simulink model "arducopter"  (R2024b)
settings: Solver=FixedStepAuto  StartTime=0.0  StopTime=simIn.param.timeEnd  FixedStep=simIn.param.dt  RelTol=1e-3
undefined symbols (not defined in the file or in its folder): DiscIntNeverNeededParam, sim, simIn
libraries: simulink x60, slident x4, vrlib x1
(part 8 of 9)

== matlab function arducopter/Rate Controller/PID Yaw Rate/Slew Limiter/Calculate Dmod ==
  data: slew_rate input; Dmod output single; sr_max input; sr_tau input; dt input; time input; pos_event_idx data_store_memory; pos_event_stored data_store_memory; pos_event_ms data_store_memory; neg_event_idx data_store_memory; neg_event_stored data_store_memory; neg_event_ms data_store_memory; modifier_slew_rate data_store_memory; output_slew_rate data_store_memory; max_neg_slew_event_ms data_store_memory; max_pos_slew_event_ms data_store_memory; max_neg_slew_rate data_store_memory; max_pos_slew_rate data_store_memory
function Dmod   = fcn(slew_rate, sr_max, sr_tau, dt, time)
% Code is based on SlewLimiter::modifier() in SlewLimiter.cpp. 

% Define global variables, so that quanitities do not have to be fed back
% to the function
global pos_event_stored;
global pos_event_idx;
global pos_event_ms;
global max_pos_slew_rate;
global max_pos_slew_event_ms;
global neg_event_stored;
global neg_event_idx;
global neg_event_ms;
global max_neg_slew_rate;
global max_neg_slew_event_ms;
global modifier_slew_rate;
global output_slew_rate;

% Definition of constants as done in SlewLimiter.h
SLEWLIMITER_N_EVENTS = uint32(3); % Number of positive and negative consecutive slew rate exceedance events recorded. Set to 3 because of 1-based indexing.
WINDOW_MS = uint32(300); % Time in ms required for half a cycle of the slowest oscillation frequency expected
MODIFIER_GAIN = 1.5; % Ratio of modifier reduction to slew rate exceedance

if (dt < 0)
    Dmod = single(1.0);
    return;
end

now_ms = uint32(time);
decay_alpha = min(dt, sr_tau) / sr_tau;

% Apply a filter to decay maximum seen slew rate once the value had left the window period
attack_alpha = min(2.0 * decay_alpha, 1.0);

%% Calculate maximum slew rate
% Save new maximum slew rates, if oldest maximum is exceeded
% OR decay the peak slew rates (pos. and neg.) if they are outside the
% observed time window
% Never drop PID gains below 10% of configured value
if (slew_rate > max_pos_slew_rate)
    max_pos_slew_rate(:) = slew_rate;
    max_pos_slew_event_ms = now_ms;
elseif (now_ms - max_pos_slew_event_ms > WINDOW_MS)
    max_pos_slew_rate = max_pos_slew_rate * (1.0 - decay_alpha);
end

if (-slew_rate > max_neg_slew_rate)
    max_neg_slew_rate(:) = -slew_rate;
    max_neg_slew_event_ms = now_ms;
elseif (now_ms - max_neg_slew_event_ms > WINDOW_MS)
    max_neg_slew_rate = max_neg_slew_rate * (1.0 - decay_alpha);
end

% Calculate the averaged maximum slew rate
raw_slew_rate = 0.5 * (max_pos_slew_rate + max_neg_slew_rate);
% Calculation of output slew rate
output_slew_rate = output_slew_rate + (raw_slew_rate - output_slew_rate) * attack_alpha;
output_slew_rate = min(raw_slew_rate, output_slew_rate);

% Check if slew limiter is activated
if(sr_max <= 0)
   Dmod = single(1.0);
   return;
end

% Constrain slew rate used for calculation
limited_raw_slew_rate = 0.5 * (min(max_pos_slew_rate, 10 * sr_max) + min(max_neg_slew_rate, 10 * sr_max));


%% Save exceedance events in event time vector
% Store a series of positive slew rate exceedance events
if (~pos_event_stored && slew_rate > sr_max)
    if (pos_event_idx >= SLEWLIMITER_N_EVENTS)
        pos_event_idx(:) = 1;
    end
    pos_event_ms(pos_event_idx) = now_ms;
    pos_event_idx(:) = pos_event_idx + 1;
    pos_event_stored = true;
    neg_event_stored = false;
end

% Store a series of negative slew rate exceedance events
if (~neg_event_stored && -slew_rate > sr_max)
    if (neg_event_idx >= SLEWLIMITER_N_EVENTS)
        neg_event_idx(:) = 1;
    end
    neg_event_ms(neg_event_idx) = now_ms;
    neg_event_idx(:) = neg_event_idx + 1;
    pos_event_stored = false;
    neg_event_stored = true;
end

% Find oldest event time
oldest_ms = now_ms;
for i=1:SLEWLIMITER_N_EVENTS-1
   oldest_ms = min(oldest_ms, pos_event_ms(i));
   oldest_ms = min(oldest_ms, neg_event_ms(i));
end

% When the oldest exceedance event falls outside of the window required for
% the number of exceedance events, apply a further reduction to the maximum
% slew rate. This prevents unwanted gain reductions caused by spikes in the
% demanded angular rates due to changed control modes or similar causes.
modifier_input = limited_raw_slew_rate;
if(now_ms - oldest_ms > SLEWLIMITER_N_EVENTS * WINDOW_MS) % no incrementation of SLEWLIMITER_N_EVENTS because of 1 based indexing
   oldest_time_from_window = single(0.001) * single(now_ms - oldest_ms - SLEWLIMITER_N_EVENTS * WINDOW_MS); 
   modifier_input = modifier_input * single(exp(-oldest_time_from_window / sr_tau));
end

%% Calculation of modifier slew rate

modifier_slew_rate = modifier_slew_rate + (modifier_input - modifier_slew_rate) * attack_alpha;
modifier_slew_rate = min(modifier_slew_rate, modifier_input);

% Calculate modifier. Only has an impact if sr_max is exceeded by averaged
% slew rate.
if(modifier_slew_rate > sr_max)
    Dmod(:) = sr_max / (sr_max + MODIFIER_GAIN * (modifier_slew_rate - sr_max));
else
    Dmod(:) = 1.0;
end

== matlab function arducopter/Position Controller/PID Velocity z/I/Integrator ==
  data: error input; integrator_out output; integrator input single; limitNeg input; limitPos input; ki input; i_max input; dt input
function integrator_out = fcn(error, integrator, limitNeg, limitPos, ki, i_max, dt)
% Code is based on AC_PID_Basic::update_i() in AC_PID_Basic.

% Check plausibility of input parameters
if (ki ~= 0)
    % Integration can only be executed if limits are not exceeded or if
    % limits are exceeded but the current error would reduce output
    if (~((limitNeg && error < 0) || (limitPos && error > 0)))
        integrator_out = integrator + error * ki * dt;
        integrator_out = max( min(integrator_out, i_max), -i_max);
    else % Otherwise, keep old integrator value
        integrator_out = integrator;
    end
else % Reset integrator if input parameters are not plausible
    integrator_out = single(0.0);
end

== matlab function arducopter/Position Controller/PID Acceleration z/I/Integrator ==
  data: error input; integrator_out output; integrator input single; limit_flg input; ki input; i_max input; dt input
function integrator_out = fcn(error, integrator, limit_flg, ki, i_max, dt)
% Code is based on AC_PID::update_i() in AC_PID, line 230.

% Check plausibility of input parameters
if (ki ~= 0 && dt > 0)
    % Only allow integration if limit is not set or the absolute sum of the
    % integrator would be reduced.
    if (~limit_flg || (integrator > 0 && error < 0) || (integrator < 0 && error > 0))
        integrator_out = integrator + error * ki * dt;
        integrator_out = min( max(integrator_out, -i_max), i_max);
    else % Otherwise, keep old integrator value
        integrator_out = integrator;
    end
else % Reset integrator if input parameters are not plausible
    integrator_out = single(0.0);
end

== matlab function arducopter/Position Controller/PID Acceleration z/Slew Limiter/Calculate Dmod ==
  data: slew_rate input; Dmod output single; sr_max input; sr_tau input; dt input; time input; pos_event_idx data_store_memory; pos_event_stored data_store_memory; pos_event_ms data_store_memory; neg_event_idx data_store_memory; neg_event_stored data_store_memory; neg_event_ms data_store_memory; modifier_slew_rate data_store_memory; output_slew_rate data_store_memory; max_neg_slew_event_ms data_store_memory; max_pos_slew_event_ms data_store_memory; max_neg_slew_rate data_store_memory; max_pos_slew_rate data_store_memory
function Dmod   = fcn(slew_rate, sr_max, sr_tau, dt, time)
% Code is based on SlewLimiter::modifier() in SlewLimiter.cpp. 

% Define global variables, so that quanitities do not have to be fed back
% to the function
global pos_event_stored;
global pos_event_idx;
global pos_event_ms;
global max_pos_slew_rate;
global max_pos_slew_event_ms;
global neg_event_stored;
global neg_event_idx;
global neg_event_ms;
global max_neg_slew_rate;
global max_neg_slew_event_ms;
global modifier_slew_rate;
global output_slew_rate;

% Definition of constants as done in SlewLimiter.h
SLEWLIMITER_N_EVENTS = uint32(3); % Number of positive and negative consecutive slew rate exceedance events recorded. Set to 3 because of 1-based indexing.
WINDOW_MS = uint32(300); % Time in ms required for half a cycle of the slowest oscillation frequency expected
MODIFIER_GAIN = 1.5; % Ratio of modifier reduction to slew rate exceedance

if (dt < 0)
    Dmod = single(1.0);
    return;
end

now_ms = uint32(time);
decay_alpha = min(dt, sr_tau) / sr_tau;

% Apply a filter to decay maximum seen slew rate once the value had left the window period
attack_alpha = min(2.0 * decay_alpha, 1.0);

%% Calculate maximum slew rate
% Save new maximum slew rates, if oldest maximum is exceeded
% OR decay the peak slew rates (pos. and neg.) if they are outside the
% observed time window
% Never drop PID gains below 10% of configured value
if (slew_rate > max_pos_slew_rate)
    max_pos_slew_rate(:) = slew_rate;
    max_pos_slew_event_ms = now_ms;
elseif (now_ms - max_pos_slew_event_ms > WINDOW_MS)
    max_pos_slew_rate = max_pos_slew_rate * (1.0 - decay_alpha);
end

if (-slew_rate > max_neg_slew_rate)
    max_neg_slew_rate(:) = -slew_rate;
    max_neg_slew_event_ms = now_ms;
elseif (now_ms - max_neg_slew_event_ms > WINDOW_MS)
    max_neg_slew_rate = max_neg_slew_rate * (1.0 - decay_alpha);
end

% Calculate the averaged maximum slew rate
raw_slew_rate = 0.5 * (max_pos_slew_rate + max_neg_slew_rate);
% Calculation of output slew rate
output_slew_rate = output_slew_rate + (raw_slew_rate - output_slew_rate) * attack_alpha;
output_slew_rate = min(raw_slew_rate, output_slew_rate);

% Check if slew limiter is activated
if(sr_max <= 0)
   Dmod = single(1.0);
   return;
end

% Constrain slew rate used for calculation
limited_raw_slew_rate = 0.5 * (min(max_pos_slew_rate, 10 * sr_max) + min(max_neg_slew_rate, 10 * sr_max));


%% Save exceedance events in event time vector
% Store a series of positive slew rate exceedance events
if (~pos_event_stored && slew_rate > sr_max)
    if (pos_event_idx >= SLEWLIMITER_N_EVENTS)
        pos_event_idx(:) = 1;
    end
    pos_event_ms(pos_event_idx) = now_ms;
    pos_event_idx(:) = pos_event_idx + 1;
    pos_event_stored = true;
    neg_event_stored = false;
end

% Store a series of negative slew rate exceedance events
if (~neg_event_stored && -slew_rate > sr_max)
    if (neg_event_idx >= SLEWLIMITER_N_EVENTS)
        neg_event_idx(:) = 1;
    end
    neg_event_ms(neg_event_idx) = now_ms;
    neg_event_idx(:) = neg_event_idx + 1;
    pos_event_stored = false;
    neg_event_stored = true;
end

% Find oldest event time
oldest_ms = now_ms;
for i=1:SLEWLIMITER_N_EVENTS-1
   oldest_ms = min(oldest_ms, pos_event_ms(i));
   oldest_ms = min(oldest_ms, neg_event_ms(i));
end

% When the oldest exceedance event falls outside of the window required for
% the number of exceedance events, apply a further reduction to the maximum
% slew rate. This prevents unwanted gain reductions caused by spikes in the
% demanded angular rates due to changed control modes or similar causes.
modifier_input = limited_raw_slew_rate;
if(now_ms - oldest_ms > SLEWLIMITER_N_EVENTS * WINDOW_MS) % no incrementation of SLEWLIMITER_N_EVENTS because of 1 based indexing
   oldest_time_from_window = single(0.001) * single(now_ms - oldest_ms - SLEWLIMITER_N_EVENTS * WINDOW_MS); 
   modifier_input = modifier_input * single(exp(-oldest_time_from_window / sr_tau));
end

%% Calculation of modifier slew rate

modifier_slew_rate = modifier_slew_rate + (modifier_input - modifier_slew_rate) * attack_alpha;
modifier_slew_rate = min(modifier_slew_rate, modifier_input);

% Calculate modifier. Only has an impact if sr_max is exceeded by averaged
% slew rate.
if(modifier_slew_rate > sr_max)
    Dmod(:) = sr_max / (sr_max + MODIFIER_GAIN * (modifier_slew_rate - sr_max));
else
    Dmod(:) = 1.0;
end

== matlab function arducopter/Motor Mixer/Calculate motor thrust ==
  data: roll input; limitRoll output; limitPitch output; pitch input; yaw input; thrIn input; thrAvgMax input; thrThstMaxIn input; compGain input; yawHeadroom input; numMotors input; facMotors input; limitYaw output; limitThrLower output; limitThrUpper output; thrOut output; thstOut output; thst_rpyt data_store_memory
function [limitRoll, limitPitch, limitYaw, limitThrLower, limitThrUpper, thrOut, thstOut] = outputArmedStabilizing(roll, pitch, yaw, thrIn, thrAvgMax, thrThstMaxIn, compGain, yawHeadroom, numMotors, facMotors)
% The calculation is taken from output_armed_stabilizing() in
% AP_MotorsMatrix.cpp.
% Contrary to the original code, lost motors are not considered

global thst_rpyt;

%% Preperations
% Definitions
roll_factor = facMotors(1,:);              % Factors of motors for thrust on differen axis - needs to moved to Init-file, together with calculation
pitch_factor = facMotors(2,:);
yaw_factor = facMotors(3,:);
throttle_factor = facMotors(4,:);
limitRoll = false;                             % Initialize limit flags to prevent missing assignment error of Simulink
limitPitch = false;
limitYaw = false;
limitThrLower = false;
limitThrUpper = false;
yaw_allowed = single(1.0);                          % Amount of yaw that can be realized
rpy_scale = single(1.0);                            % Scale factor to fit roll, pitch and yaw within motor limits
throttle_thrust_best_rpy = single(0.0);             % Amount of throttle that provides maximum roll, pitch and yaw without climbing                      
thrust_boost_ratio = single(0.0);                   % Ratio for thrust boosting in case of a motor failure. Set to 0 for normal operation!     

% TODO: Voltage and air pressure compensation
roll_thrust = roll * compGain;
pitch_thrust = pitch * compGain;
yaw_thrust = yaw * compGain;
throttle_thrust = thrIn * compGain;             % Pilot's desired throttle
thrAvgMax = thrAvgMax * compGain;

% Calculate maximum throttle thrust input value
throttle_thrust_max = thrust_boost_ratio + (1.0 - thrust_boost_ratio) * thrThstMaxIn;

% Sanity check: Throttle above zero and below current limnited throttle.
% Limit Throttle otherwise
if (throttle_thrust <= 0)
    throttle_thrust = single(0.0);
    limitThrLower = true;
end
if (throttle_thrust >= throttle_thrust_max)
    throttle_thrust = throttle_thrust_max;
    limitThrUpper = true;
end
% Limit throttle average max
thrAvgMax = max( min( thrAvgMax, throttle_thrust_max), throttle_thrust);
% Calculate highest allowed average throttle that will provide maximum
% control range of roll, pitch and yaw without climbing
throttle_thrust_best_rpy = min(single(0.5), thrAvgMax);

%% Calculation of the throttle that gives most room for yaw
% This corresponds to the lower of
%   1. 0.5 - (rpy_low + rpy_high) / 2.0) --> This gives the maximum
%   possible margin above the highest motor and below the lowest
%   2. The higher of
%       a) Pilots throttle input
%       b) The point throttle_rpy_mix between pilot's input throttle and
%       hover throttle

% First: Calculate amount of yaw that fits into throttle range
% amount of yaw we can fit in
yaw_allowed = single(1.0);
for i=1:numMotors
    % Combined thrust output of roll and pitch
    thst_rpyt(i) = roll_thrust * roll_factor(i) + pitch_thrust * pitch_factor(i); 
    
    % % Record lowest thrust command
    % if (thst_rpyt(i) < rp_low)
    %     rp_low = thst_rpyt(i);
    % end
    % % Record highest thrust command
    % if (thst_rpyt(i) > rp_high)
    %     rp_high = thst_rpyt(i);
    % end
    
    % Check maximum yaw control that can be used
    if(yaw_factor(i)~=0)
        thrust_rp_best_throttle = throttle_thrust_best_rpy + thst_rpyt(i);
        if ((yaw_thrust * yaw_factor(i)) > 0)
           motor_room = 1 - thrust_rp_best_throttle;
        else
           motor_room = thrust_rp_best_throttle;
        end
        motor_yaw_allowed = max(motor_room, 0) / abs(yaw_factor(i));
        yaw_allowed = min(yaw_allowed, motor_yaw_allowed);
    end    
end

% Calculate the maximum yaw control that can be used
yaw_allowed_min = yawHeadroom / 1000.0;
% If thrust boost is enabled, increase headroom to 50%
yaw_allowed_min = thrust_boost_ratio * 0.5 + (1.0 - thrust_boost_ratio) * yaw_allowed_min;

yaw_allowed = max(yaw_allowed, yaw_allowed_min);

%% Add yaw control to thrust outputs
% Limit yaw thrust to allowed range
if (abs(yaw_thrust) > yaw_allowed)
    yaw_thrust = min( max(-yaw_allowed, yaw_thrust), yaw_allowed);
    limitYaw = true;
end

rpy_low = single(1.0);
rpy_high = single(-1.0);
for i=1:numMotors
    % Combined thrust command for roll, pitch and yaw
   thst_rpyt(i) = thst_rpyt(i) + yaw_thrust * yaw_factor(i);
   
   % Record lowest thrust command
    if (thst_rpyt(i) < rpy_low)
        rpy_low = thst_rpyt(i);
    end
    % Record highest thrust command
    if (thst_rpyt(i) > rpy_high)
        rpy_high = thst_rpyt(i);
    end
end

%% Scale outputs
% Calculate any sclaing that is needed to fit combined thrust outputs
% within the output range
if (rpy_high - rpy_low > 1.0)
    rpy_scale(:) = 1.0 / (rpy_high-rpy_low);
end
if (thrAvgMax + rpy_low < 0)
    rpy_scale(:) = min(rpy_scale, -thrAvgMax / rpy_low);
end

% Calculate how close the motors can come to the desired throttle
rpy_high = rpy_high * rpy_scale;
rpy_low = rpy_low * rpy_scale;
throttle_thrust_best_rpy = -rpy_low;
% Calculate the difference between pilot's desired throttle and
% throttle_thrust_best_rpy
thr_adj = single(throttle_thrust - throttle_thrust_best_rpy);
if (rpy_scale < 1.0) % Full range of throttle is already being used
    limitRoll(:) = true;
    limitPitch(:) = true;
    limitYaw(:) = true;
    if (thr_adj > 0.0)
       limitThrUpper = true; 
    end
    thr_adj(:) = 0.0;
else
    if (thr_adj < 0.0) % Throttle can't be reduced to reach desired value
        thr_adj(:) = 0.0;
    elseif (thr_adj > 1.0 - (throttle_thrust_best_rpy + rpy_high))
       % Throttle can't be increased to desired value
       thr_adj(:) = 1.0 - (throttle_thrust_best_rpy + rpy_high);
       limitThrUpper = true;
    end
end

%% Calculate resulting thrust outputs
% Calculate adjusted throttle value
throttle_thrust_best_plus_adj = throttle_thrust_best_rpy + thr_adj;
% Add scaled roll, pitch, constrained yaw and throttle for each motor
for i=1:numMotors
    % Combined thrust is the sum of the maximum possible desired throttle
    % "throttle_thrust_best_plus_adj" and the needed thrust to realize the
    % desired angular motion "thrust_rpyt_out(i)"
    thst_rpyt(i) = (throttle_thrust_best_plus_adj * throttle_factor(i)) + (rpy_scale * thst_rpyt(i)); 
end

% Calculate throttle thrust after mixing for harmonic notch
thrOut = throttle_thrust_best_plus_adj / compGain;

% Assign thrust output
thstOut = thst_rpyt;

== matlab function arducopter/Position Controller/P Position z/Calculate error ==
  settings: updateMethod=DISCRETE
  data: tar input; tar_new output; err output; act input; err_min input; err_max input
function [tar_new, err] = calc_err(tar, act, err_min, err_max)
% Code based on AC_P_1D::update_all() in AC_P_1D.cpp.
tar_new = tar; % added line to prevent Simulink error for unassigned tar_new
err = tar - act;

% Limit error and recalculate target
if ((err_min < 0) && (err < err_min))
    err = err_min;
    tar_new = act + err;
elseif ((err_max > 0) && (err > err_max))
    err = err_max;
    tar_new = act + err;
end

== matlab function arducopter/Position Controller/P Position z/Set vertical speed & acceleration limit/Set error limits ==
  data: outMin input; errMin output; outMax input; DoutMax input; errMax output; D1max output; D2OutMax input; kp input
function [errMin, errMax, D1max] = setLimits(outMin, outMax, DoutMax, D2OutMax, kp)
% Code taken from AC_P_1D::set_limits() in AC_P_1D.cpp.
% Input parameter D2_out_max is neglected since it is set to zero in
% AC_PosControl::set_correction_speed_accel_z()

errMin = single(0.0);
errMax = single(0.0);
D1max = single(0.0);

if (DoutMax > 0)
   D1max = DoutMax; 
end

% Missing line left out because of parameter D2_out_max being set to 0

% Call the simulink function inv_sqrt_controller(...) from control.cpp,
% line 343 if the conditions apply
if (outMin < 0 && kp > 0)
    errMin = inv_sqrt_controller(outMin, kp, DoutMax);
end

if (outMax > 0 && kp > 0)
    errMax = inv_sqrt_controller(outMax, kp, DoutMax);
end

== matlab function arducopter/Position Controller/P Position z/Set vertical speed & acceleration limit/Inverse Square Root Controller/Inverse Sqrt Controller ==
  data: output input; errLim output; p input; Dmax input
function errLim = inv_sqrt_controller(output, p, Dmax)
% Code taken from inv_sqrt_controller(...) in control.cpp.
% Function calculates the input (error) to the sqrt_controller required to
% achieve a given output

if (Dmax > 0 && p == 0)
    errLim = output * output / (single(2.0) * Dmax);
    return;
end
if ((Dmax < 0 || Dmax == 0) && p ~= 0)
    errLim = output / p;
    return;
end
if ((Dmax < 0 || Dmax == 0) && p == 0)
   errLim = single(0.0);
   return
end

% Calculate the cross-point velocity, at which we switch from calculating the
% controller output using a linear function to a sqrt function
linear_velocity = Dmax / p;
% Use linear function to calculate limit if current velocity is below
% cross-point velocity
if (abs(output) < linear_velocity)
   errLim = output / p;
   return;
end

% Calculate the cross-point distance at which we switch to sqrt function
linear_dist = Dmax / (p*p);
% Calculate the maximum distance error resulting from the velocity and
% acceleration limit
stopping_dist = (linear_dist * single(0.5)) + (output*output) / (single(2.0) * Dmax);
% If output parameter is negative or zero, return negative maximum distance
% error
if (output > 0)
    errLim = stopping_dist;
else
    errLim = -stopping_dist;
end

== matlab function arducopter/Position Controller/P Position z/Square Root Controller ==
  data: err input; correction_rate output; p input; second_ord_lim input; dt input
function correction_rate = sqrt_controller(err, p, second_ord_lim, dt)
% The square root controller
% Code is taken from sqrt_controller(...) in AC_PosControl.cpp.

if (second_ord_lim < 0 || second_ord_lim == 0)
   correction_rate = err * p;
elseif (p == 0)
    % P term is zero, but second order limit is positive
    if (err > 0)
        correction_rate = sqrt(single(2.0) * second_ord_lim * err);
    elseif (err < 0)
        correction_rate = sqrt(single(2.0) * second_ord_lim * -err);
    else
        correction_rate = single(0.0);
    end
else
    % P term and second order limit are positive, hence have been defined
    linear_dist = second_ord_lim / (p * p);
    % Check if error exceeds linear range of controller gain
    if (err > linear_dist)
        correction_rate = sqrt(single(2.0) * second_ord_lim * ( err - (linear_dist / single(2.0)) ));
    elseif (err < -linear_dist)
        correction_rate = -sqrt(single(2.0) * second_ord_lim * ( -err - (linear_dist / single(2.0)) ));
    else
        % Return linearly amplified correction if error is in linear range
        correction_rate = err * p;
    end
end

% Prevent oscillations by over-shooting the error correction in the last
% time step
if (dt > 0)
    correction_rate = min( max(correction_rate, -abs(err) / dt), abs(err) / dt);
end

== matlab function arducopter/Position Controller/PID Acceleration z/Slew Limiter/Lowpass Filter ==
  data: in input; out output single; alpha input; out_last input
function out  = apply(in, alpha, out_last)
% The code is based on the apply(sample, cutoff_freq, dt) function in
% LowPassFilter.cpp

% Output calculation
out = out_last + (in - out_last) * alpha;

== matlab function arducopter/Throttle/Throttle Calculations/Throttle-Attitude-Mixing/Update Throttle Mix Des ==
  data: thrTar input; zVelCtrlRatio input; zVelDes input; thrMan input; thrMixDes output; thrMixMin input; thrMixMax input; thrMixMan input
function thrMixDes = updateThrottleMix(thrTar, zVelCtrlRatio, zVelDes, thrMan, thrMixMin, thrMixMax, thrMixMan)
% Sets desired throttle vs attitude priorization based on vehicle state.
% Low values favour pilot/autopilot throttle over attitude control, high
% values favour attitude control over throttle
% Has not effect when throttle > hover throttle
% Code: land_detector.cpp, Copter::update_throttle_mix()

if thrMan
    % Manual throttle
    if thrTar <= 0
        % Call to set_throttle_mix_min() set mix to minimum
        thrMixDes = thrMixMin;
    else
        % Call to set_throttle_mix_man() sets mix to value for manual
        % throttle
        thrMixDes = thrMixMan;
    end
else
    % Autopilot controlled throttle
    
    % Check for aggressive flight request - Requested roll/pitch angle
    % above 15 degrees
    % ToDo

    % Check for large external disturbances - angle error over 30 degrees
    % ToDo

    % Check for large acceleration - falling for high turbulence
    % ToDo

    % Check for requested descent
    descent_not_demanded = zVelDes >= single(0.0);

    if (descent_not_demanded)
        % Call to AC_AttitudeControl_Multi::set_throttle_mix_max(ratio)
        ratio = min( max(single(0.0), zVelCtrlRatio), single(1.0) );
        thrMixDes = (single(1.0) - ratio) * thrMixMin + ratio * thrMixMax;
    else
        thrMixDes = thrMixMin;
    end
end

== matlab function arducopter/Position Controller/zVelCtrlRatio Calculation/Update vel_z_ctrl_ratio ==
  data: velErr input; zVelCtrlRat output; dnVelMax input; dt input; vel_z_ctrl_ratio data_store_memory
function zVelCtrlRat = setZVelCtrlRatio(velErr, dnVelMax, dt)
% Sets vel_z_control_ratio, which contains the proportion of the z velocity
% error relative to the maximum request. Needed in function
% Copter::update_throttle_mix().
% Code: AC_PosControl.cpp, update_z_controller()

global vel_z_ctrl_ratio;

err_ratio = velErr / dnVelMax;
vel_z_ctrl_ratio = vel_z_ctrl_ratio + dt * single(0.1) * (0.5 - err_ratio);
vel_z_ctrl_ratio = min( max(single(0.0), vel_z_ctrl_ratio), single(2.0) );

zVelCtrlRat = vel_z_ctrl_ratio;

== matlab function arducopter/Position Controller/Vertical Speed and Acceleration Limits ==
  data: dnSpeedMax input; upSpeedMax input; zAccMax input; vel_max_down_cms data_store_memory; vel_max_up_cms data_store_memory; acc_max_z_cmss data_store_memory; jerk_max_z_cmsss data_store_memory; zJerkMax input; GRAVITY_MSS input; zAccFltt_f input; zAccFlte_f input
function setMaxSpeedAccelZ(dnSpeedMax, upSpeedMax, zAccMax, zJerkMax, GRAVITY_MSS, zAccFltt_f, zAccFlte_f)
% Sets the maximum vertical speed in cm/s and acceleration in cm/s/s.
% Checks max vertical jerk limits.
% Code: AC_PosControl.cpp, set_max_speed_accel_z().

global vel_max_down_cms;
global vel_max_up_cms;
global acc_max_z_cmss;
global jerk_max_z_cmsss;

% Make sure maximum descending speed is negative
dnSpeedMax = dnSpeedMax * single(-1);

% Sanity check
if dnSpeedMax < 0
    vel_max_down_cms = dnSpeedMax;
end
if upSpeedMax > 0
    vel_max_up_cms = upSpeedMax;
end
if zAccMax > 0
    acc_max_z_cmss = zAccMax;
end

% Ensure that vertical jerk is not limited by filter of z acceleration PID
jerk_max_z_cmsss = single(100) * zJerkMax;
if (zAccFltt_f > 0)
    jerk_max_z_cmsss = min( jerk_max_z_cmsss, min(GRAVITY_MSS * single(100), acc_max_z_cmss) * (2*pi*zAccFltt_f) / single(5.0) );
end
if (zAccFlte_f > 0)
    jerk_max_z_cmsss = min( jerk_max_z_cmsss, min(GRAVITY_MSS * single(100), acc_max_z_cmss) * (2*pi*zAccFlte_f) / single(5.0) );
end

== matlab function arducopter/Lowpass2p/Lowpass Pitch/Lowpass2p ==
  data: sample input; y output; sampleFreq input; cutoffFreq input; delElem1 data_store_memory; delElem2 data_store_memory
function y = lowpass2p(sample, sampleFreq, cutoffFreq)
% Lowpass filter of order two
% Source: LowPassFilter2p.cpp
global delElem1
global delElem2

% Calculate parameters: LowPassFilter2p.cpp, compute_params()
% Keep well under Nyquist limit
cutoffFreq = min(cutoffFreq, sampleFreq * 0.4);
fr = single(sampleFreq/cutoffFreq);
ohm = single(tan(pi/fr));
c = single(1+2*cos(pi/4)*ohm + ohm*ohm);

b0 = ohm*ohm/c;
b1 = 2*b0;
b2 = b0;
a1 = 2*(ohm*ohm-1)/c;
a2 = single((1-2*cos(pi/4)*ohm+ohm*ohm)/c);

% Calculation of filtered sample: LowPassFilter2p.cpp, apply()
if (cutoffFreq <= 0 || sampleFreq <= 0)
    y = sample;
    return;
end

delElem0 = sample - delElem1 * a1 - delElem2 * a2;
y = delElem0 * b0 + delElem1 * b1 + delElem2 * b2;

delElem2 = delElem1;
delElem1 = delElem0;

== matlab function arducopter/Lowpass2p/Lowpass Roll/Lowpass2p ==
  data: sample input; y output; sampleFreq input; cutoffFreq input; delElem1 data_store_memory; delElem2 data_store_memory
function y = lowpass2p(sample, sampleFreq, cutoffFreq)
% Lowpass filter of order two
% Source: LowPassFilter2p.cpp
global delElem1
global delElem2

% Calculate parameters: LowPassFilter2p.cpp, compute_params()
% Keep well under Nyquist limit
cutoffFreq = min(cutoffFreq, sampleFreq * 0.4);
fr = single(sampleFreq/cutoffFreq);
ohm = single(tan(pi/fr));
c = single(1+2*cos(pi/4)*ohm + ohm*ohm);

b0 = ohm*ohm/c;
b1 = 2*b0;
b2 = b0;
a1 = 2*(ohm*ohm-1)/c;
a2 = single((1-2*cos(pi/4)*ohm+ohm*ohm)/c);

% Calculation of filtered sample: LowPassFilter2p.cpp, apply()
if (cutoffFreq <= 0 || sampleFreq <= 0)
    y = sample;
    return;
end

delElem0 = sample - delElem1 * a1 - delElem2 * a2;
y = delElem0 * b0 + delElem1 * b1 + delElem2 * b2;

delElem2 = delElem1;
delElem1 = delElem0;

== matlab function arducopter/Lowpass2p/Lowpass Yaw/Lowpass2p ==
  data: sample input; y output; sampleFreq input; cutoffFreq input; delElem1 data_store_memory; delElem2 data_store_memory
function y = lowpass2p(sample, sampleFreq, cutoffFreq)
% Lowpass filter of order two
% Source: LowPassFilter2p.cpp
global delElem1
global delElem2

% Calculate parameters: LowPassFilter2p.cpp, compute_params()
% Keep well under Nyquist limit
cutoffFreq = min(cutoffFreq, sampleFreq * 0.4);
fr = single(sampleFreq/cutoffFreq);
ohm = single(tan(pi/fr));
c = single(1+2*cos(pi/4)*ohm + ohm*ohm);

b0 = ohm*ohm/c;
b1 = 2*b0;
b2 = b0;
a1 = 2*(ohm*ohm-1)/c;
a2 = single((1-2*cos(pi/4)*ohm+ohm*ohm)/c);

% Calculation of filtered sample: LowPassFilter2p.cpp, apply()
if (cutoffFreq <= 0 || sampleFreq <= 0)
    y = sample;
    return;
end

delElem0 = sample - delElem1 * a1 - delElem2 * a2;
y = delElem0 * b0 + delElem1 * b1 + delElem2 * b2;

delElem2 = delElem1;
delElem1 = delElem0;

== matlab function arducopter/Body Frame Rates -> DCM/MATLAB Function ==
  data: dcm input; quaternion output
function quaternion = from_rotation_matrix(dcm)
% Function to calculate quaternion from a given rotation matrix.
% Implemented based on QuaternionT<T>::from_rotation_matrx()

m00 = dcm(1,1);
m11 = dcm(2,2);
m22 = dcm(3,3);
m10 = dcm(2,1);
m01 = dcm(1,2);
m20 = dcm(3,1);
m02 = dcm(1,3);
m21 = dcm(3,2);
m12 = dcm(2,3);

tr = m00 + m11 + m22;

if tr > 0
    S = sqrt(tr+1) * 2;
    qw = 0.25 * S;
    qx = (m21 - m12) / S;
    qy = (m02 - m20) / S;
    qz = (m10 - m01) / S;
elseif ((m00 > m11) && (m00 > m22))
    S = sqrt(1.0 + m00 - m11 - m22) * 2.0;
    qw = (m21 - m12) / S;
    qx = 0.25 * S;
    qy = (m01 + m10) / S;
    qz = (m02 + m20) / S;
elseif (m11 > m22)
    S = sqrt(1.0 + m11 - m00 - m22) * 2.0;
    qw = (m02 - m20) / S;
    qx = (m01 + m10) / S;
    qy = 0.25 * S;
    qz = (m12 + m21) / S;
else
    S = sqrt(1.0 + m22 - m00 - m11) * 2.0;
    qw = (m10 - m01) / S;
    qx = (m02 + m20) / S;
    qy = (m12 + m21) / S;
    qz = 0.25 * S;
end

quaternion = [qw;qx;qy;qz];

== matlab function arducopter/Attitude Controller/MATLAB Function ==
  data: rollIn input; rollOut output; pitchIn input; angleMax input; angleLimit input; pitchOut output; rpyInputMax input
function [rollOut, pitchOut] = get_pilot_desired_lean_angles(rollIn, pitchIn, angleMax, angleLimit, rpyInputMax)
% Code based on Mode::get_pilot_desired_lean_angles()
% Transform pilot's roll and pitch input into desired lean angle in
% centi-degrees

% Calculate inputs to rc_input_to_roll_pitch() function
rollInUnit = rollIn / rpyInputMax;
pitchInUnit = pitchIn / rpyInputMax;
angleMax = angleMax / 100;
angleLimit = angleLimit / 100;

%% The following lines result from the call to rc_input_to_roll_pitch() (control.cpp)
angleMaxDeg = min(angleMax, 85);
rc2rad = angleMaxDeg * pi / 180;

% Convert roll and pitch stick positions to normalized horizontal thrust
thrust_x = -1 * tan(rc2rad * pitchInUnit);
thrust_y = tan(rc2rad * rollInUnit);

% Calculate the horizontal thrust limit based on the angle limit
angleLimit = min( max( 10, angleLimit), angleMaxDeg);
thrustLimit = tan(angleLimit * pi / 180);

% Apply horizontal thrust limit - Lines are taken from
% Vector2<T>::limit_length() and limit thrust vector norm
thrustVecLength = sqrt(thrust_x^2 + thrust_y^2);
if thrustVecLength > thrustLimit && thrustVecLength > 0
   thrust_x = thrust_x * (thrustLimit / thrustVecLength);
   thrust_y = thrust_y * (thrustLimit / thrustVecLength);
end

% Conversion from angular thrust to euler angles
pitchRad = (-1) * atan(thrust_x);
rollRad = atan(cos(pitchRad) * thrust_y);

% Output values in centi-degrees
pitchOut = pitchRad * (100 * 180) / pi;
rollOut = rollRad * (100 * 180) / pi;

== matlab function arducopter/Attitude Controller/MATLAB Function1 ==
  data: yawIn input; yawOut output; pilotYawExpo input; pilotYawRate input
function yawOut = get_pilot_desired_yaw_rate(yawIn, pilotYawExpo, pilotYawRate)
% Code taken from Mode::get_pilot_desired_yaw_rate()
% Transforms pilot's yaw input into a desired yaw rate

%% 1) Apply expo - Code based on input_expo in control.cpp
yawIn = min(max(yawIn, -1), 1);
if pilotYawExpo < 0.95
    yawIn = (1 - pilotYawExpo) * yawIn / (1 - pilotYawExpo * abs(yawIn));
end

%% 2) Convert pilot input to the desired yaw rate
yawOut = pilotYawRate * 100 * yawIn;

== matlab function arducopter/Attitude Controller/input_euler_angle_roll_pitch_euler_rate_yaw()/MATLAB Function ==
  data: q input; roll output; pitch output; yaw output
function [roll, pitch, yaw] = toEuler(q)
% Function takes a quaternion and translates it into Euler angles
% Based on QuaternionT<T>::to_euler() and incorporates 
% QuaternionT<T>::get_euler_roll(), QuaternionT<T>::get_euler_pitch() and
% QuaternionT<T>::get_euler_yaw()

roll = single(atan2(2 * (q(1)*q(2) + q(3)*q(4)), 1 - 2*(q(2)*q(2) + q(3)*q(3))));
% Check if argument of asin is greater than 1 oder smaller than -1
% Based on safe_asin() in AP_MATH.cpp
xPitch = 2 * (q(1)*q(3) - q(4)*q(2));
if xPitch >= 1
    pitch = single(pi/2);
elseif xPitch <= -1
    pitch = single(-pi/2);
else
    pitch = single(asin(xPitch));
end
yaw = single(atan2(2*(q(1)*q(4) + q(2)*q(3)), 1 - 2*(q(3)*q(3) + q(4)*q(4))));

== matlab function arducopter/Attitude Controller/input_euler_angle_roll_pitch_euler_rate_yaw()/Feedforward enabled/MATLAB Function ==
  data: eulerAngleTar input; eulerAccelMaxBF output; eulerAccelMaxEF input
function eulerAccelMaxBF = euler_accel_limit(eulerAngleTar, eulerAccelMaxEF)
% Translation of acceleration limits eulerAccelMax to the euler axis
% Code based on AC_AttitudeControl::euler_accel_limit()

eulerAccelMaxBF = single(zeros(3,1));
if eulerAccelMaxEF(1) < 0 || eulerAccelMaxEF(2) < 0 || eulerAccelMaxEF(3) < 0 
    eulerAccelMaxBF = eulerAccelMaxEF;
end


sin_phi = max(min(abs(single(sin(eulerAngleTar(1)))), 1), 0.1); % Sinus of roll angle
cos_phi = max(min(abs(single(cos(eulerAngleTar(1)))), 1), 0.1);
sin_theta = max(min(abs(single(sin(eulerAngleTar(2)))), 1), 0.1); % Sinus of pitch angle
cos_theta = max(min(abs(single(cos(eulerAngleTar(2)))), 1), 0.1);


eulerAccelMaxBF(1) = eulerAccelMaxEF(1);
eulerAccelMaxBF(2) = min(eulerAccelMaxEF(2) / cos_phi, eulerAccelMaxEF(3) / sin_phi);
eulerAccelMaxBF(3) = min(min(eulerAccelMaxEF(1) / sin_theta, eulerAccelMaxEF(2) / (sin_phi * cos_theta)), eulerAccelMaxEF(3) / (cos_phi * cos_theta));

== matlab function arducopter/Attitude Controller/input_euler_angle_roll_pitch_euler_rate_yaw()/Feedforward enabled/input shaping/input shaping roll angle/Square Root Controller ==
  data: err input; correction_rate output; p input; second_ord_lim input; dt input
function correction_rate = sqrt_controller(err, p, second_ord_lim, dt)
% The square root controller
% Code is taken from sqrt_controller(...) in AC_PosControl.cpp, line 296.

if (second_ord_lim < 0 || second_ord_lim == 0)
   correction_rate = err * p;
elseif (p == 0)
    % P term is zero, but second order limit is positive
    if (err > 0)
        correction_rate = sqrt(single(2.0) * second_ord_lim * err);
    elseif (err < 0)
        correction_rate = sqrt(single(2.0) * second_ord_lim * -err);
    else
        correction_rate = single(0.0);
    end
else
    % P term and second order limit are positive, hence have been defined
    linear_dist = second_ord_lim / (p * p);
    % Check if error exceeds linear range of controller gain
    if (err > linear_dist)
        correction_rate = sqrt(single(2.0) * second_ord_lim * ( err - (linear_dist / single(2.0)) ));
    elseif (err < -linear_dist)
        correction_rate = -sqrt(single(2.0) * second_ord_lim * ( -err - (linear_dist / single(2.0)) ));
    else
        % Return linearly amplified correction if error is in linear range
        correction_rate = err * p;
    end
end

% Prevent oscillations by over-shooting the error correction in the last
% time step
if (dt ~= 0)
    correction_rate = max( min(correction_rate, abs(err) / dt), -abs(err) / dt);
end

== matlab function arducopter/Attitude Controller/input_euler_angle_roll_pitch_euler_rate_yaw()/Feedforward enabled/input shaping/input shaping roll angle/MATLAB Function ==
  data: radIn input; radLim output
function radLim = wrapPi(radIn)
% Function to limit input angle in radian to [-pi pi].
% Code based on wrap_PI() and wrap_2PI() of AP_Math.cpp

% 1) Limit to [0 2pi]
radLim = mod(radIn, 2*pi);
if radLim < 0
    radLim = radLim + 2*pi;
end

% 2) Limit to [0 pi]
if radLim > pi
    radLim = radLim - 2*pi;
end

== matlab function arducopter/Attitude Controller/input_euler_angle_roll_pitch_euler_rate_yaw()/Feedforward enabled/input shaping/input shaping roll angle/MATLAB Function1 ==
  data: desiredAngVel input; targetAngVel input; eulerRateTar output; accelMax input; dt input; input_tc input
function eulerRateTar = input_shaping_ang_vel(desiredAngVel, targetAngVel, accelMax, dt, input_tc)
% Limits acceleration and deceleration of a velocity request
% Code based on AC_AttitudeControl::input_shaping_ang_vel()

if input_tc > 0
    % Calculate the acceleration to smoothly achieve rate. Jerk is not limited.
    errorRate = desiredAngVel - targetAngVel;
    desiredAngAccel = sqrt_controller(errorRate, 1.0/max(input_tc, single(0.01)), single(0), dt);
    desiredAngVel = targetAngVel + desiredAngAccel * dt;
end

% Acceleration is limited directly to smooth the beginning of the curve
if accelMax > 0
    deltaAngVel = accelMax * dt;
    eulerRateTar = min(max(desiredAngVel, targetAngVel - deltaAngVel), targetAngVel + deltaAngVel);
else
    eulerRateTar = desiredAngVel;
end

== matlab function arducopter/Attitude Controller/input_euler_angle_roll_pitch_euler_rate_yaw()/Feedforward enabled/input shaping/input shaping pitch angle/MATLAB Function ==
  data: radIn input; radLim output
function radLim = wrapPi(radIn)
% Function to limit input angle in radian to [-pi pi].
% Code based on wrap_PI() and wrap_2PI() of AP_Math.cpp

% 1) Limit to [0 2pi]
radLim = mod(radIn, 2*pi);
if radLim < 0
    radLim = radLim + 2*pi;
end

% 2) Limit to [0 pi]
if radLim > pi
    radLim = radLim - 2*pi;
end

== matlab function arducopter/Attitude Controller/input_euler_angle_roll_pitch_euler_rate_yaw()/reset yaw targets/MATLAB Function9 ==
  data: q1 input; qRes output; q2 input
function qRes = quatMult(q1, q2)
% Quaternion multiplication. Code based on QuaternionT<T>::operator*() in
% quaternion.cpp

qRes = single(zeros(4,1));
qRes(1) = q1(1)*q2(1) - q1(2)*q2(2) - q1(3)*q2(3) - q1(4)*q2(4);
qRes(2) = q1(1)*q2(2) + q1(2)*q2(1) + q1(3)*q2(4) - q1(4)*q2(3);
qRes(3) = q1(1)*q2(3) - q1(2)*q2(4) + q1(3)*q2(1) + q1(4)*q2(2);
qRes(4) = q1(1)*q2(4) + q1(2)*q2(3) - q1(3)*q2(2) + q1(4)*q2(1);

== matlab function arducopter/Attitude Controller/input_euler_angle_roll_pitch_euler_rate_yaw()/Feedforward enabled/input shaping/input shaping pitch angle/Square Root Controller ==
  data: err input; correction_rate output; p input; second_ord_lim input; dt input
function correction_rate = sqrt_controller(err, p, second_ord_lim, dt)
% The square root controller
% Code is taken from sqrt_controller(...) in AC_PosControl.cpp, line 296.

if (second_ord_lim < 0 || second_ord_lim == 0)
   correction_rate = err * p;
elseif (p == 0)
    % P term is zero, but second order limit is positive
    if (err > 0)
        correction_rate = sqrt(single(2.0) * second_ord_lim * err);
    elseif (err < 0)
        correction_rate = sqrt(single(2.0) * second_ord_lim * -err);
    else
        correction_rate = single(0.0);
    end
else
    % P term and second order limit are positive, hence have been defined
    linear_dist = second_ord_lim / (p * p);
    % Check if error exceeds linear range of controller gain
    if (err > linear_dist)
        correction_rate = sqrt(single(2.0) * second_ord_lim * ( err - (linear_dist / single(2.0)) ));
    elseif (err < -linear_dist)
        correction_rate = -sqrt(single(2.0) * second_ord_lim * ( -err - (linear_dist / single(2.0)) ));
    else
        % Return linearly amplified correction if error is in linear range
        correction_rate = err * p;
    end
end

% Prevent oscillations by over-shooting the error correction in the last
% time step
if (dt ~= 0)
    correction_rate = max( min(correction_rate, abs(err) / dt), -abs(err) / dt);
end

== matlab function arducopter/Rate Controller/PID Pitch Rate/I/Integrator ==
  data: error input; integrator_out output; integrator input single; limit_flg input; ki input; i_max input; dt input
function integrator_out = fcn(error, integrator, limit_flg, ki, i_max, dt)
% Code is based on AC_PID::update_i() in AC_PID.cpp.

% Check plausibility of input parameters
if (ki ~= 0 && dt > 0)
    % Only allow integration if limit is not set or the absolute sum of the
    % integrator would be reduced.
    if (~limit_flg || (integrator > 0 && error < 0) || (integrator < 0 && error > 0))
        integrator_out = integrator + error * ki * dt;
        integrator_out = max( min(integrator_out, i_max), -i_max);
    else % Otherwise, keep old integrator value
        integrator_out = integrator;
    end
else % Reset integrator if input parameters are not plausible
    integrator_out = single(0.0);
end

== matlab function arducopter/Attitude Controller/input_euler_angle_roll_pitch_euler_rate_yaw()/Feedforward enabled/MATLAB Function1 ==
  data: eulerAngle input; angVelTar output; eulerRate input
function angVelTar = euler_rate_to_ang_vel(eulerAngle, eulerRate)
% This function converts euler angle derivatives (321 system) to an angular
% velocity vector. eulerAngle is the vector of the euler angles in rad and
% eulerRate is the vector of euler rates in rad/s
% Code based on AC_AttitudeControl::euler_rate_to_ang_vel()

sin_theta = single(sin(eulerAngle(2)));
cos_theta = single(cos(eulerAngle(2)));
sin_phi = single(sin(eulerAngle(1)));
cos_phi = single(cos(eulerAngle(1)));

angVelTar = single(zeros(3,1));
angVelTar(1) = eulerRate(1) - sin_theta * eulerRate(3);
angVelTar(2) = cos_phi * eulerRate(2) + sin_phi * cos_theta * eulerRate(3);
angVelTar(3) = -sin_phi * eulerRate(2) + cos_theta * cos_phi * eulerRate(3);

== matlab function arducopter/Attitude Controller/input_euler_angle_roll_pitch_euler_rate_yaw()/reset yaw targets/MATLAB Function1 ==
  data: q input; roll output; pitch output; yaw output
function [roll, pitch, yaw] = toEuler(q)
% Function takes a quaternion and translates it into Euler angles
% Based on QuaternionT<T>::to_euler() and incorporates 
% QuaternionT<T>::get_euler_roll(), QuaternionT<T>::get_euler_pitch() and
% QuaternionT<T>::get_euler_yaw()

roll = single(atan2(2 * (q(1)*q(2) + q(3)*q(4)), 1 - 2*(q(2)*q(2) + q(3)*q(3))));
% Check if argument of asin is greater than 1 oder smaller than -1
% Based on safe_asin() in AP_MATH.cpp
xPitch = 2 * (q(1)*q(3) - q(4)*q(2));
if xPitch >= 1
    pitch = single(pi/2);
elseif xPitch <= -1
    pitch = single(-pi/2);
else
    pitch = single(asin(xPitch));
end
yaw = single(atan2(2*(q(1)*q(4) + q(2)*q(3)), 1 - 2*(q(3)*q(3) + q(4)*q(4))));

== matlab function arducopter/Attitude Controller/input_euler_angle_roll_pitch_euler_rate_yaw()/Feedforward enabled/MATLAB Function2 ==
  data: angVelTar input; angVelTarLimited output; angVelRollMax input; angVelPitchMax input; angVelYawMax input
function angVelTarLimited = ang_vel_limit(angVelTar, angVelRollMax, angVelPitchMax, angVelYawMax)
% Limits angular velocity (rad/s) in body frame
% Code based on AC_AttitudeControl::ang_vel_limit()

angVelTarLimited = angVelTar;
if angVelRollMax == 0 || angVelPitchMax == 0
    if angVelRollMax ~= 0
        angVelTarLimited(1) = max(min(angVelTar(1), angVelRollMax), -angVelRollMax);
    end
    if angVelPitchMax ~= 0
        angVelTarLimited(2) = max(min(angVelTar(2), angVelPitchMax), -angVelPitchMax);
    end
else
    thrustVecAngVel = [angVelTar(1) / angVelRollMax; angVelTar(2) / angVelPitchMax];
    thrustVecLen = single(sqrt(thrustVecAngVel(1)^2 + thrustVecAngVel(2)^2));
    if thrustVecLen > 1
        angVelTarLimited(1) = thrustVecAngVel(1) * angVelRollMax / thrustVecLen;
        angVelTarLimited(2) = thrustVecAngVel(2) * angVelPitchMax / thrustVecLen;
    end
end
if angVelYawMax ~= 0
    angVelTarLimited(3) = max(min(angVelTar(3), angVelYawMax), -angVelYawMax);
end

== matlab function arducopter/Attitude Controller/input_euler_angle_roll_pitch_euler_rate_yaw()/Feedforward enabled/MATLAB Function3 ==
  data: angVelBf input; eulerAngle input; eulerRate output
function eulerRate = ang_vel_to_euler_rate(angVelBf,eulerAngle)
% Function converts body-frame angular velocity into euler rate of desired
% attitude
% Based on AC_AttitudeControl::ang_vel_to_euler_rate()

sin_theta = single(sin(eulerAngle(2)));
cos_theta = single(cos(eulerAngle(2)));
sin_phi = single(sin(eulerAngle(1)));
cos_phi = single(cos(eulerAngle(1)));

eulerRate = single(zeros(3,1));
eulerRate(1) = angVelBf(1) + sin_phi * (sin_theta / cos_theta) * angVelBf(2) + cos_phi * (sin_theta / cos_theta) * angVelBf(3);
eulerRate(2) = cos_phi * angVelBf(2) - sin_phi * angVelBf(3);
eulerRate(3) = (sin_phi / cos_theta) * angVelBf(2) + (cos_phi / cos_theta) * angVelBf(3);

== matlab function arducopter/Attitude Controller/input_euler_angle_roll_pitch_euler_rate_yaw()/Feedforward disabled/MATLAB Function ==
  data: roll input; q output; pitch input; yaw input
function q = fromEuler(roll, pitch, yaw)
% Computes quaternion from euler angle vector
% Based on QuaternionT<T>::from_euler()

q = single(zeros(4,1));
cr2 = single(cos(roll*0.5));
cp2 = single(cos(pitch*0.5));
cy2 = single(cos(yaw*0.5));
sr2 = single(sin(roll*0.5));
sp2 = single(sin(pitch*0.5));
sy2 = single(sin(yaw*0.5));

q(1) = cr2*cp2*cy2 + sr2*sp2*sy2;
q(2) = sr2*cp2*cy2 - cr2*sp2*sy2;
q(3) = cr2*sp2*cy2 + sr2*cp2*sy2;
q(4) = cr2*cp2*sy2 - sr2*sp2*cy2;

== matlab function arducopter/Attitude Controller/input_euler_angle_roll_pitch_euler_rate_yaw()/thrust_heading_rotation_angles()/thrust_vector_rotation_angles()/MATLAB Function ==
  data: q input; vecRot output; vec input
function vecRot = rotateByQuat(q, vec)
% Function rotates vector vec by quaternion q. Equivalent to converting the
% input quaternion to a rotation matrix and then multiplying it by the
% vector. This uses the formula
%
%    v2 = v1 + 2 q1 * qv x v1 + 2 qv x qv x v1
%
% where "x" is the cross product (explicitly inlined for performance below), 
% "q1" is the scalar part and "qv" is the vector part of this quaternion
% Code based on Vector3<T> QuaternionT<T>::operator*()

vecRot = vec;

% Compute and cache "qv x v1"
uv = [q(3) * vec(3) - q(4) * vec(2); q(4) * vec(1) - q(2) * vec(3); q(2) * vec(2) - q(3) * vec(1)];

uv(1) = uv(1) + uv(1);
uv(2) = uv(2) + uv(2);
uv(3) = uv(3) + uv(3);
vecRot(1) = vecRot(1) + q(1) * uv(1) + q(3) * uv(3) - q(4) * uv(2);
vecRot(2) = vecRot(2) + q(1) * uv(2) + q(4) * uv(1) - q(2) * uv(3);
vecRot(3) = vecRot(3) + q(1) * uv(3) + q(2) * uv(2) - q(3) * uv(1);

== matlab function arducopter/Attitude Controller/input_euler_angle_roll_pitch_euler_rate_yaw()/thrust_heading_rotation_angles()/thrust_vector_rotation_angles()/MATLAB Function1 ==
  data: q input; vecRot output; vec input
function vecRot = rotateByQuat(q, vec)
% Function rotates vector vec by quaternion q. Equivalent to converting the
% input quaternion to a rotation matrix and then multiplying it by the
% vector. This uses the formula
%
%    v2 = v1 + 2 q1 * qv x v1 + 2 qv x qv x v1
%
% where "x" is the cross product (explicitly inlined for performance below), 
% "q1" is the scalar part and "qv" is the vector part of this quaternion
% Code based on Vector3<T> QuaternionT<T>::operator*()

vecRot = vec;

% Compute and cache "qv x v1"
uv = [q(3) * vec(3) - q(4) * vec(2); q(4) * vec(1) - q(2) * vec(3); q(2) * vec(2) - q(3) * vec(1)];

uv(1) = uv(1) + uv(1);
uv(2) = uv(2) + uv(2);
uv(3) = uv(3) + uv(3);
vecRot(1) = vecRot(1) + q(1) * uv(1) + q(3) * uv(3) - q(4) * uv(2);
vecRot(2) = vecRot(2) + q(1) * uv(2) + q(4) * uv(1) - q(2) * uv(3);
vecRot(3) = vecRot(3) + q(1) * uv(3) + q(2) * uv(2) - q(3) * uv(1);
